simulink model "afe_rst_inv_psm_distributed_control_two_delays"  (R2026a)
settings: Solver=ode1be  StopTime=simlength  FixedStep=tc  MaxStep=Tc
values from neighbouring files (symbols this model uses):
  Amplitude_U = 1.16    [grid_fault_generator.m]
  Amplitude_V = Amplitude_U    (= 1.16)    [grid_fault_generator.m]
  Amplitude_W = Amplitude_U    (= 1.16)    [grid_fault_generator.m]
  end_time_LVRT = start_time_LVRT + error_length    [grid_fault_generator.m]
  Igrid_phase_normalization_factor = 270*sqrt(2)    [grid_emulator.m]
  omega_grid_emulator_nom = w_grid    (= 314.159265359)    [grid_emulator.m]
  omega_grid_nom = w_grid    (= 314.159265359)    [grid_emulator.m]
  t_ramp = 20e-3    (= 0.02)    [grid_fault_generator.m]
  ugrid_factor = 1    [grid_emulator.m]
  V_phase_normalization_factor = Vgrid_phase_normalization_factor    [grid_emulator.m]
  Vdc_bez = 1070    [grid_emulator.m]
  Vemu_ref_norm = Vemu_ref * sqrt(2) / V_phase_normalization_factor    [grid_emulator.m]
  vn_eta_pu = 0    [grid_emulator.m]
  vn_xi_pu = 0    [grid_emulator.m]
  vp_xi_pu = 1    [grid_emulator.m]
undefined symbols (not defined in the file or in its folder): Adrso, Aresd, Bresd, CFi, CFu, Cresd, Crso, CTRPIFF_CLIP_RELEASE, dead_time_INV, emf_fb_p, emf_fb_p_ccaller_1, emf_fb_p_ccaller_2, emf_p, emf_p_ccaller_1, emf_p_ccaller_2, fPWM_INV, g0_161Hz, g0_500Hz, g1_161Hz, g1_500Hz, i_grid_neg_eta_lim, i_grid_neg_eta_red_lim, i_grid_neg_xi_lim, i_grid_neg_xi_red_lim, i_grid_pos_eta_lim, i_grid_pos_eta_red_lim, ibez, id_lim, ieta_neg_ref_lim, ieta_pos_ref_lim, iq_lim, ixi_pos_ref_lim, Jm_norm, k_frt_ref, kg, ki_afe, ki_i, ki_id, ki_iq, ki_rc_neg_grid, ki_rc_pos_grid, ki_vs, ki_w, kp_afe, kp_i, kp_id, kp_iq, kp_rc_neg_grid, kp_rc_pos_grid, kp_vs, kp_w, kw, l1, l2, Lalpha_norm, Ld_norm, Ldrso, Lq_norm, Ls_norm, luenberger_l1 ... (+30)
libraries: fl_lib x146, nesl_utility x62, simulink x8, cstblocks_lti x7, sl_discontinuities x3, single_phase_transformer_lib x3, flexshaft_lib x1, permanent_magnet_synchronous_machine x1
(part 7 of 14)

== system afe_rst_inv_psm_distributed_control_two_delays/INV-Modular/inv_leg_w/driver_board_w/double_integrator_observer ==
  theta : Inport
  Gain : Gain  Gain=kw
  Gain1 : Gain  Gain=kg
  Gain4 : Gain  Gain=omega_bez
  Gain5 : Gain  Gain=ts_inv
  Gain6 : Gain  Gain=1/omega_bez
  Sum : Sum  Inputs=-+|
  Sum1 : Sum  Inputs=|++
  Sum2 : Sum  Inputs=|++
  Sum8 : Sum  Inputs=++|
  Unit Delay1 : UnitDelay  SampleTime=ts_inv
  Unit Delay2 : UnitDelay  SampleTime=ts_inv
  bounder1 : MATLAB Function  TreatAsAtomicUnit=on  SystemSampleTime=ts_inv
  bounder2 : MATLAB Function  TreatAsAtomicUnit=on  SystemSampleTime=ts_inv
  omega_pu_hat : Outport  VectorParamsAs1DForOutWhenUnconnected=off
  theta_hat : Outport  Port=2  VectorParamsAs1DForOutWhenUnconnected=off
  wires:
  theta/1 -> Sum/2  "theta"
  Sum8/1 -> bounder2/1(u)
  Sum1/1 -> Unit Delay2/1
  Unit Delay2/1 -> omega_pu_hat/1, Sum1/2, Gain5/1
  Sum2/1 -> Sum8/2
  bounder2/1(y) -> Unit Delay1/1
  bounder1/1(y) -> Gain/1, Gain1/1
  Gain5/1 -> Gain4/1
  Sum/1 -> bounder1/1(u)
  Unit Delay1/1 -> Sum2/2, theta_hat/1, Sum/1  "theta_hat"
  Gain/1 -> Gain6/1
  Gain6/1 -> Sum1/1
  Gain4/1 -> Sum8/1
  Gain1/1 -> Sum2/1

== system afe_rst_inv_psm_distributed_control_two_delays/INV-Modular/inv_leg_w/driver_board_w/motor_vector_control ==
  motor_torque_ref : Inport
  Bus Creator1 : BusCreator  Inputs=2
  Unit Delay2 : UnitDelay  SampleTime=ts_inv
  Unit Delay3 : UnitDelay  SampleTime=ts_inv
  Variant Source : VariantSource  VariantControls={use_psm_encoder == 1, use_psm_encoder == 0}
  bemf_observer : Subsystem
  current_ctrl : Subsystem
  current_transformation : Subsystem
  dq2alphabeta : MATLAB Function  TreatAsAtomicUnit=on  SystemSampleTime=ts_inv
  us_alphabeta_ctrl : Outport
  tag scope: motor_ualpha_ctrl_dbw=global, motor_ubeta_ctrl_dbw=global
  wires:
  [isv_pu_dbv_fb_dbw] -> current_transformation/2(v)
  Bus Creator1/1 -> us_alphabeta_ctrl/1
  motor_torque_ref/1 -> current_ctrl/1(iq_ref)  "motor_torque_ref"
  dq2alphabeta/2(beta) -> Unit Delay3/1
  [motor_ibeta_pu_dbu] -> bemf_observer/2(ibeta_pu)
  [motor_ubeta_ctrl_dbw] -> Bus Creator1/2  "motor_ubeta_ctrl"
  [isu_pu_dbu_fb_dbw] -> current_transformation/1(u)
  [motor_ualpha_ctrl_dbw] -> Bus Creator1/1  "motor_ualpha_ctrl"
  [motor_ualpha_ctrl_dbu] -> bemf_observer/3(ualpha_pu)
  [motor_ubeta_ctrl_dbu] -> bemf_observer/4(ubeta_pu)
  [motor_ialpha_pu_dbu] -> bemf_observer/1(ialpha_pu)
  current_ctrl/1(ud) -> dq2alphabeta/1(d)
  current_ctrl/2(uq) -> dq2alphabeta/2(q)
  Unit Delay2/1 -> [motor_ualpha_ctrl_dbw]
  [isw_pu_dbw] -> current_transformation/3(w)
  Variant Source/1 -> current_transformation/4(gamma), dq2alphabeta/3(gamma)
  dq2alphabeta/1(alpha) -> Unit Delay2/1
  Unit Delay3/1 -> [motor_ubeta_ctrl_dbw]
  [motor_theta_hat_dbw] -> Variant Source/2
  [motor_phase_mb_fb_dbw_luenberger] -> Variant Source/1

== system afe_rst_inv_psm_distributed_control_two_delays/INV-Modular/inv_leg_w/driver_board_w/voltage-current-acquisition ==
  From3 : From  Commented=on  GotoTag=usu_ctrl_dbu  TagVisibility=global
  From4 : From  Commented=on  GotoTag=usv_ctrl_dbv  TagVisibility=global
  Goto6 : Goto  Commented=on  GotoTag=usu_ctrl_dbu_fb_dbw  TagVisibility=global
  Goto7 : Goto  Commented=on  GotoTag=usv_ctrl_dbv_fb_dbw  TagVisibility=global
  isu_fieldbus : Subsystem
  isv_fieldbus : Subsystem
  isw_measure_and_normalization : Subsystem
  motor_phase_fieldbus : Subsystem
  motor_torque_fieldbus : Subsystem
  usu_ctrl_fieldbus : Subsystem  Commented=on
  usu_fieldbus : Subsystem
  usv_ctrl_fieldbus : Subsystem  Commented=on
  usv_fieldbus : Subsystem
  usw_measure_and_normalization : Subsystem
  tag scope: isu_pu_dbu_fb_dbw=global, isv_pu_dbv_fb_dbw=global, isw_pu_dbw=global, motor_phase_mb_fb_dbw=global, motor_torque_ref_dbu_fb_dbw=global, usu_pu_dbu_fb_dbw=global, usv_pu_dbv_fb_dbw=global, usw_pu_dbw=global
  wires:
  usu_fieldbus/1(us_fb) -> [usu_pu_dbu_fb_dbw]
  usv_fieldbus/1(us_fb) -> [usv_pu_dbv_fb_dbw]
  [usu_pu_dbu] -> usu_fieldbus/1(us)
  [usv_pu_dbv] -> usv_fieldbus/1(us)
  usw_measure_and_normalization/1(us_pu) -> [usw_pu_dbw]
  [usw_dbw] -> usw_measure_and_normalization/1(us)
  isv_fieldbus/1(is_fb) -> [isv_pu_dbv_fb_dbw]
  usv_ctrl_fieldbus/1(u_ctrl_fb) -> Goto7/1
  [isw_dbw] -> isw_measure_and_normalization/1(is)
  From3/1 -> usu_ctrl_fieldbus/1(u_ctrl)
  [isu_pu_dbu] -> isu_fieldbus/1(is)
  isw_measure_and_normalization/1(is_pu) -> [isw_pu_dbw]
  From4/1 -> usv_ctrl_fieldbus/1(u_ctrl)
  isu_fieldbus/1(is_fb) -> [isu_pu_dbu_fb_dbw]
  [isv_pu_dbv] -> isv_fieldbus/1(is)
  usu_ctrl_fieldbus/1(u_ctrl_fb) -> Goto6/1
  motor_torque_fieldbus/1(motor_torque_ref_fb) -> [motor_torque_ref_dbu_fb_dbw]
  [motor_torque_ref_dbu] -> motor_torque_fieldbus/1(motor_torque_ref)
  motor_phase_fieldbus/1(motor_phase_fb) -> [motor_phase_mb_fb_dbw]
  [motor_phase_mb] -> motor_phase_fieldbus/1(motor_phase)

== system afe_rst_inv_psm_distributed_control_two_delays/INV-Modular/inv_leg_w/modulator/sv_pwm ==
  u_alphabeta_ctrl : Inport
  enable : Inport  Port=2
  Bus Selector : BusSelector  OutputSignals=dc
  Bus Selector1 : BusSelector  OutputSignals=motor_ualpha_ctrl,motor_ubeta_ctrl
  C Caller : CCaller  FunctionName=sv_pwm_process_simulink  PortSpecificationStruct="%)30     .    N @   8    (     @         %    \"     4    !     0         %  0 \"0    $    _    07)G3F%M90  4&]R=$YA;64 4V-O<&4     26YD97@     5'EP90      4VEZ90      27-';&]B86P   X    P    !@    @    $          4    (     0    ,    !         !   P!O=70 #@   #     &    \"     0         !0    @    !     P    $         $  # &]U=  .    .     8    (    !          %    \"     $    &     0         0   ...(+2630 chars)"  SampleTime=ts_inv
  Constant : Constant  Value=ts_inv
  Data Type Conversion15 : DataTypeConversion  OutDataTypeStr=single  SaturateOnIntegerOverflow=off  RndMeth=Floor
  Data Type Conversion16 : DataTypeConversion  OutDataTypeStr=single  SaturateOnIntegerOverflow=off  RndMeth=Floor
  Data Type Conversion17 : DataTypeConversion  OutDataTypeStr=uint32  SaturateOnIntegerOverflow=off  RndMeth=Floor
  Data Type Conversion18 : DataTypeConversion  OutDataTypeStr=single  SaturateOnIntegerOverflow=off  RndMeth=Floor
  Data Type Conversion3 : DataTypeConversion  OutDataTypeStr=double  SaturateOnIntegerOverflow=off  RndMeth=Floor
  Zero-Order Hold{,1..3} (4 alike) : ZeroOrderHold  SampleTime=ts_inv
  modulator : Subsystem
  firing_gates : Outport
  wires:
  Bus Selector/1 -> Data Type Conversion3/1  "<dc>"
  Data Type Conversion3/1 -> modulator/1(w)  "dw"
  Bus Selector1/2 -> Data Type Conversion15/1  "<motor_ubeta_ctrl>"
  Bus Selector1/1 -> Data Type Conversion18/1  "<motor_ualpha_ctrl>"
  u_alphabeta_ctrl/1 -> Bus Selector1/1
  modulator/1(firing_gates) -> firing_gates/1
  C Caller/1 -> Bus Selector/1  "out"
  Data Type Conversion15/1 -> Zero-Order Hold1/1
  Zero-Order Hold3/1 -> C Caller/4
  Data Type Conversion17/1 -> Zero-Order Hold3/1
  Zero-Order Hold1/1 -> C Caller/2
  Data Type Conversion16/1 -> Zero-Order Hold2/1
  enable/1 -> Data Type Conversion17/1
  Data Type Conversion18/1 -> Zero-Order Hold/1
  Constant/1 -> Data Type Conversion16/1
  Zero-Order Hold2/1 -> C Caller/3
  Zero-Order Hold/1 -> C Caller/1

== system afe_rst_inv_psm_distributed_control_two_delays/INV-Modular/inv_leg_w/solid_state_inverter/switch_1 ==
  Diode : fl_lib/Electrical/Electrical Elements/Diode  Vf=Vgamma V  Ron=Ron Ohm  Goff=1e-8 1/Ohm  i_specify=off  i_priority=None  i=0 A  i_nominal_specify=off  i_nominal_value=1  i_nominal_unit=A  v_specify=off  v_priority=None  v=0 V  v_nominal_specify=off  v_nominal_value=1  v_nominal_unit=V
  Switch : fl_lib/Electrical/Electrical Elements/Switch  R_closed=Ron Ohm  G_open=1e-8 1/Ohm  Threshold=7.5  i_specify=off  i_priority=None  i=0 A  i_nominal_specify=off  i_nominal_value=1  i_nominal_unit=A  v_specify=off  v_priority=None  v=0 V  v_nominal_specify=off  v_nominal_value=1  v_nominal_unit=V
  snubber : fl_lib/Electrical/Electrical Elements/Capacitor  c=Csnubber F  r=Rsnubber Ohm  g=0 1/Ohm  i_specify=off  i_priority=None  i=0 A  i_nominal_specify=off  i_nominal_value=1  i_nominal_unit=A  v_specify=off  v_priority=None  v=0 V  v_nominal_specify=off  v_nominal_value=1  v_nominal_unit=V  vc_specify=off  vc_priority=High  vc=0 V  vc_nominal_specify=off  vc_nominal_value=1  vc_nominal_unit=V
  G : PMIOPort  Side=Left
  C : PMIOPort  Port=2  Side=Left
  E : PMIOPort  Port=3  Side=Right
  connections:
  Diode/LConn1 -- snubber/RConn1 -- E/RConn1 -- Switch/LConn1
  Switch/RConn1 -- G/RConn1
  Diode/RConn1 -- snubber/LConn1 -- C/RConn1 -- Switch/RConn2

== system afe_rst_inv_psm_distributed_control_two_delays/INV-Modular/inv_leg_w/solid_state_inverter/switch_2 ==
  Diode : fl_lib/Electrical/Electrical Elements/Diode  Vf=Vgamma V  Ron=Ron Ohm  Goff=1e-8 1/Ohm  i_specify=off  i_priority=None  i=0 A  i_nominal_specify=off  i_nominal_value=1  i_nominal_unit=A  v_specify=off  v_priority=None  v=0 V  v_nominal_specify=off  v_nominal_value=1  v_nominal_unit=V
  Switch : fl_lib/Electrical/Electrical Elements/Switch  R_closed=Ron Ohm  G_open=1e-8 1/Ohm  Threshold=7.5  i_specify=off  i_priority=None  i=0 A  i_nominal_specify=off  i_nominal_value=1  i_nominal_unit=A  v_specify=off  v_priority=None  v=0 V  v_nominal_specify=off  v_nominal_value=1  v_nominal_unit=V
  snubber : fl_lib/Electrical/Electrical Elements/Capacitor  c=Csnubber F  r=Rsnubber Ohm  g=0 1/Ohm  i_specify=off  i_priority=None  i=0 A  i_nominal_specify=off  i_nominal_value=1  i_nominal_unit=A  v_specify=off  v_priority=None  v=0 V  v_nominal_specify=off  v_nominal_value=1  v_nominal_unit=V  vc_specify=off  vc_priority=High  vc=0 V  vc_nominal_specify=off  vc_nominal_value=1  vc_nominal_unit=V
  G : PMIOPort  Side=Left
  C : PMIOPort  Port=2  Side=Left
  E : PMIOPort  Port=3  Side=Right
  connections:
  Diode/RConn1 -- snubber/LConn1 -- Switch/RConn2 -- C/RConn1
  Switch/RConn1 -- G/RConn1
  Diode/LConn1 -- snubber/RConn1 -- Switch/LConn1 -- E/RConn1

== system afe_rst_inv_psm_distributed_control_two_delays/grid/grid_emulator/grid_emulator/phase_gen ==
  Constant4 : Constant  Value=omega_grid_emulator_nom
  Integrator : Integrator
  To Workspace7 : ToWorkspace  VariableName=gamma_grid_emulator_sim  SampleTime=ts_afe
      settings: MaxDataPoints=Ns_afe
  bounder1 : MATLAB Function  TreatAsAtomicUnit=on  SystemSampleTime=ts_afe
  grid_emu_phase : Outport  VectorParamsAs1DForOutWhenUnconnected=off
  tag scope: gamma_grid_emulator=global
  wires:
  bounder1/1(y) -> [gamma_grid_emulator], To Workspace7/1, grid_emu_phase/1  "grid_emu_phase"
  Constant4/1 -> Integrator/1
  Integrator/1 -> bounder1/1(u)

== system afe_rst_inv_psm_distributed_control_two_delays/grid/grid_emulator/grid_emulator/voltage_reference ==
  grid_emu_phase : Inport
  Vxi_p : Inport  Port=2
  Vxi_n : Inport  Port=3
  Veta_n : Inport  Port=4
  Constant2 : Constant  Value=0
  Grid: Voltage-Source in abc : Subsystem
  Manual Switch : ManualSwitch  CurrentSetting=0
  Manual Switch1 : ManualSwitch  CurrentSetting=0
  Manual Switch2 : ManualSwitch  CurrentSetting=0
  Sum1 : Sum  Inputs=|++
  Sum4 : Sum  Inputs=|++
  alphabeta2abc : MATLAB Function  TreatAsAtomicUnit=on  SystemSampleTime=ts_afe
  xieta2alphabeta_neg : MATLAB Function  TreatAsAtomicUnit=on  SystemSampleTime=ts_afe
  xieta2alphabeta_pos : MATLAB Function  TreatAsAtomicUnit=on  SystemSampleTime=ts_afe
  V1_ref1 : Outport  VectorParamsAs1DForOutWhenUnconnected=off
  V2_ref1 : Outport  Port=2  VectorParamsAs1DForOutWhenUnconnected=off
  V3_ref1 : Outport  Port=3  VectorParamsAs1DForOutWhenUnconnected=off
  wires:
  xieta2alphabeta_pos/1(alpha) -> Sum1/1
  Sum1/1 -> alphabeta2abc/1(alpha)
  xieta2alphabeta_pos/2(beta) -> Sum4/1
  Sum4/1 -> alphabeta2abc/2(beta)
  xieta2alphabeta_neg/1(alpha) -> Sum1/2
  xieta2alphabeta_neg/2(beta) -> Sum4/2
  grid_emu_phase/1 -> Grid: Voltage-Source in abc/1(gamma), xieta2alphabeta_neg/3(gamma), xieta2alphabeta_pos/3(gamma)
  Vxi_p/1 -> xieta2alphabeta_pos/1(xi)
  Constant2/1 -> xieta2alphabeta_pos/2(eta)
  Vxi_n/1 -> xieta2alphabeta_neg/1(xi)
  Veta_n/1 -> xieta2alphabeta_neg/2(eta)
  alphabeta2abc/1(a) -> [V1_ref_xieta]
  alphabeta2abc/2(b) -> [V2_ref_xieta]
  alphabeta2abc/3(c) -> [V3_ref_xieta]
  [V3_ref_abc] -> Manual Switch2/2
  Manual Switch2/1 -> V3_ref1/1
  [V2_ref_abc] -> Manual Switch1/2
  Manual Switch/1 -> V1_ref1/1
  Grid: Voltage-Source in abc/1(vp_xi) -> [V1_ref_abc]
  Grid: Voltage-Source in abc/2(vn_xi) -> [V2_ref_abc]
  Grid: Voltage-Source in abc/3(vn_eta) -> [V3_ref_abc]
  [V1_ref_abc] -> Manual Switch/2
  [V1_ref_xieta] -> Manual Switch/1
  [V2_ref_xieta] -> Manual Switch1/1
  Manual Switch1/1 -> V2_ref1/1
  [V3_ref_xieta] -> Manual Switch2/1

== system afe_rst_inv_psm_distributed_control_two_delays/grid/grid_emulator/grid_emulator/voltage_source ==
  Constant : Constant  Value=vp_xi_pu
  Constant1 : Constant  Value=vn_xi_pu
  Constant2 : Constant  Value=vn_eta_pu
  Gain1 : Gain  Gain=V_phase_normalization_factor
  Gain2 : Gain  Gain=ugrid_factor
  Gain3 : Gain  Gain=ugrid_factor
  Gain4 : Gain  Gain=ugrid_factor
  Gain7 : Gain  Gain=V_phase_normalization_factor
  Gain8 : Gain  Gain=V_phase_normalization_factor
  LTI System3 : cstblocks_lti/LTI System  sys=LVRT_flt_ss_c  IC=[]  PadeOrder=0
  LTI System4 : cstblocks_lti/LTI System  sys=LVRT_flt_ss_c  IC=[]  PadeOrder=0
  LTI System5 : cstblocks_lti/LTI System  sys=LVRT_flt_ss_c  IC=[]  PadeOrder=0
  vp_xi : Outport  VectorParamsAs1DForOutWhenUnconnected=off
  vn_xi : Outport  Port=2  VectorParamsAs1DForOutWhenUnconnected=off
  vn_eta : Outport  Port=3  VectorParamsAs1DForOutWhenUnconnected=off
  wires:
  LTI System3/1 -> Gain7/1
  LTI System4/1 -> Gain8/1
  Gain7/1 -> Gain2/1
  Gain8/1 -> Gain3/1
  Gain1/1 -> Gain4/1
  LTI System5/1 -> Gain1/1
  Gain2/1 -> vp_xi/1
  Gain3/1 -> vn_xi/1
  Gain4/1 -> vn_eta/1
  Constant2/1 -> LTI System5/1
  Constant1/1 -> LTI System4/1
  Constant/1 -> LTI System3/1

== system afe_rst_inv_psm_distributed_control_two_delays/grid/instantaneus_power/abc2alphabeta/abc2alphabeta ==
  a : Inport
  b : Inport  Port=2
  c : Inport  Port=3
  Gain1 : Gain  Gain=-1/2
  Gain11 : Gain  Gain=-1/2
  Gain2 : Gain  Gain=0
  Gain3 : Gain  Gain=sqrt(3)/2
  Gain4 : Gain  Gain=-sqrt(3)/2
  Gain8 : Gain  Gain=2/3
  Gain9 : Gain  Gain=2/3
  Sum : Sum  Inputs=+++
  Sum1 : Sum  Inputs=+++
  "alpha " : Outport  VectorParamsAs1DForOutWhenUnconnected=off
  "beta " : Outport  Port=2  VectorParamsAs1DForOutWhenUnconnected=off
  wires:
  Gain11/1 -> Sum/2
  Gain1/1 -> Sum/3
  Gain9/1 -> "beta "/1
  Gain8/1 -> "alpha "/1
  Gain2/1 -> Sum1/1
  Gain3/1 -> Sum1/2
  Gain4/1 -> Sum1/3
  a/1 -> Gain2/1, Sum/1
  c/1 -> Gain4/1, Gain1/1
  b/1 -> Gain3/1, Gain11/1
  Sum/1 -> Gain8/1
  Sum1/1 -> Gain9/1

== system afe_rst_inv_psm_distributed_control_two_delays/grid/instantaneus_power/abc2alphabeta /abc->alphabeta ==
  a : Inport
  b : Inport  Port=2
  c : Inport  Port=3
  Gain1 : Gain  Gain=-1/2
  Gain11 : Gain  Gain=-1/2
  Gain2 : Gain  Gain=0
  Gain3 : Gain  Gain=sqrt(3)/2
  Gain4 : Gain  Gain=-sqrt(3)/2
  Gain8 : Gain  Gain=2/3
  Gain9 : Gain  Gain=2/3
  Sum : Sum  Inputs=+++
  Sum1 : Sum  Inputs=+++
  "alpha " : Outport  VectorParamsAs1DForOutWhenUnconnected=off
  "beta " : Outport  Port=2  VectorParamsAs1DForOutWhenUnconnected=off
  wires:
  Sum1/1 -> Gain9/1
  Sum/1 -> Gain8/1
  b/1 -> Gain11/1, Gain3/1
  c/1 -> Gain1/1, Gain4/1
  a/1 -> Sum/1, Gain2/1
  Gain4/1 -> Sum1/3
  Gain3/1 -> Sum1/2
  Gain2/1 -> Sum1/1
  Gain8/1 -> "alpha "/1
  Gain9/1 -> "beta "/1
  Gain1/1 -> Sum/3
  Gain11/1 -> Sum/2

== system afe_rst_inv_psm_distributed_control_two_delays/mainboard_afe/current_sequence_avg/Moving Average Filter5/Enabled Subsystem ==
  In1 : Inport
  Enable : EnablePort
  Constant2 : Constant
  Divide : Product  Inputs=*/
  Gain1 : Gain  Gain=1/(2*pi)
  Gain9 : Gain  Gain=2
  Zero-Order Hold : ZeroOrderHold  SampleTime=ts_afe
  Out1 : Outport
  wires:
  Gain1/1 -> Gain9/1
  Zero-Order Hold/1 -> Out1/1  "period"
  Gain9/1 -> Divide/2
  In1/1 -> Gain1/1  "Omega_el"
  Divide/1 -> Zero-Order Hold/1
  Constant2/1 -> Divide/1

== system afe_rst_inv_psm_distributed_control_two_delays/mainboard_afe/current_sequence_avg/Moving Average Filter5/Reset Trigger ==
  Clock : Clock
  Constant1 : Constant  Value=simlength
  Constant3 : Constant  Value=0
  Constant4 : Constant
  Mod : Math  Operator=mod
  Switch : Switch  Criteria=u2 ~= 0  SaturateOnIntegerOverflow=off  InputSameDT=off
  Zero-Order Hold : ZeroOrderHold  SampleTime=ts_afe
  Out1 : Outport
  wires:
  Constant1/1 -> Mod/2
  Switch/1 -> Out1/1  "Reset"
  Clock/1 -> Zero-Order Hold/1
  Mod/1 -> Switch/2
  Constant4/1 -> Switch/3
  Zero-Order Hold/1 -> Mod/1
  Constant3/1 -> Switch/1

== system afe_rst_inv_psm_distributed_control_two_delays/mainboard_afe/current_sequence_avg/Moving Average Filter6/Enabled Subsystem ==
  In1 : Inport
  Enable : EnablePort
  Constant2 : Constant
  Divide : Product  Inputs=*/
  Gain1 : Gain  Gain=1/(2*pi)
  Gain9 : Gain  Gain=2
  Zero-Order Hold : ZeroOrderHold  SampleTime=ts_afe
  Out1 : Outport
  wires:
  Constant2/1 -> Divide/1
  Divide/1 -> Zero-Order Hold/1
  In1/1 -> Gain1/1  "Omega_el"
  Gain9/1 -> Divide/2
  Zero-Order Hold/1 -> Out1/1  "period"
  Gain1/1 -> Gain9/1

== system afe_rst_inv_psm_distributed_control_two_delays/mainboard_afe/current_sequence_avg/Moving Average Filter6/Reset Trigger ==
  Clock : Clock
  Constant1 : Constant  Value=simlength
  Constant3 : Constant  Value=0
  Constant4 : Constant
  Mod : Math  Operator=mod
  Switch : Switch  Criteria=u2 ~= 0  SaturateOnIntegerOverflow=off  InputSameDT=off
  Zero-Order Hold : ZeroOrderHold  SampleTime=ts_afe
  Out1 : Outport
  wires:
  Constant3/1 -> Switch/1
  Zero-Order Hold/1 -> Mod/1
  Constant4/1 -> Switch/3
  Mod/1 -> Switch/2
  Clock/1 -> Zero-Order Hold/1
  Switch/1 -> Out1/1  "Reset"
  Constant1/1 -> Mod/2

== system afe_rst_inv_psm_distributed_control_two_delays/mainboard_afe/current_sequence_avg/Moving Average Filter7/Enabled Subsystem ==
  In1 : Inport
  Enable : EnablePort
  Constant2 : Constant
  Divide : Product  Inputs=*/
  Gain1 : Gain  Gain=1/(2*pi)
  Gain9 : Gain  Gain=2
  Zero-Order Hold : ZeroOrderHold  SampleTime=ts_afe
  Out1 : Outport
  wires:
  Gain1/1 -> Gain9/1
  Zero-Order Hold/1 -> Out1/1  "period"
  Gain9/1 -> Divide/2
  In1/1 -> Gain1/1  "Omega_el"
  Divide/1 -> Zero-Order Hold/1
  Constant2/1 -> Divide/1

== system afe_rst_inv_psm_distributed_control_two_delays/mainboard_afe/current_sequence_avg/Moving Average Filter7/Reset Trigger ==
  Clock : Clock
  Constant1 : Constant  Value=simlength
  Constant3 : Constant  Value=0
  Constant4 : Constant
  Mod : Math  Operator=mod
  Switch : Switch  Criteria=u2 ~= 0  SaturateOnIntegerOverflow=off  InputSameDT=off
  Zero-Order Hold : ZeroOrderHold  SampleTime=ts_afe
  Out1 : Outport
  wires:
  Constant1/1 -> Mod/2
  Switch/1 -> Out1/1  "Reset"
  Clock/1 -> Zero-Order Hold/1
  Mod/1 -> Switch/2
  Constant4/1 -> Switch/3
  Zero-Order Hold/1 -> Mod/1
  Constant3/1 -> Switch/1

== system afe_rst_inv_psm_distributed_control_two_delays/mainboard_afe/current_sequence_avg/Moving Average Filter8/Enabled Subsystem ==
  In1 : Inport
  Enable : EnablePort
  Constant2 : Constant
  Divide : Product  Inputs=*/
  Gain1 : Gain  Gain=1/(2*pi)
  Gain9 : Gain  Gain=2
  Zero-Order Hold : ZeroOrderHold  SampleTime=ts_afe
  Out1 : Outport
  wires:
  Constant2/1 -> Divide/1
  Divide/1 -> Zero-Order Hold/1
  In1/1 -> Gain1/1  "Omega_el"
  Gain9/1 -> Divide/2
  Zero-Order Hold/1 -> Out1/1  "period"
  Gain1/1 -> Gain9/1

== system afe_rst_inv_psm_distributed_control_two_delays/mainboard_afe/current_sequence_avg/Moving Average Filter8/Reset Trigger ==
  Clock : Clock
  Constant1 : Constant  Value=simlength
  Constant3 : Constant  Value=0
  Constant4 : Constant
  Mod : Math  Operator=mod
  Switch : Switch  Criteria=u2 ~= 0  SaturateOnIntegerOverflow=off  InputSameDT=off
  Zero-Order Hold : ZeroOrderHold  SampleTime=ts_afe
  Out1 : Outport
  wires:
  Constant3/1 -> Switch/1
  Zero-Order Hold/1 -> Mod/1
  Constant4/1 -> Switch/3
  Mod/1 -> Switch/2
  Clock/1 -> Zero-Order Hold/1
  Switch/1 -> Out1/1  "Reset"
  Constant1/1 -> Mod/2

== system afe_rst_inv_psm_distributed_control_two_delays/mainboard_afe/dq_pll/pll_stageA/abc_to_alphabeta ==
  ug_a : Inport
  ug_b : Inport  Port=2
  ug_c : Inport  Port=3
  abc2alphabeta : MATLAB Function  TreatAsAtomicUnit=on  SystemSampleTime=ts_afe
  ug_alpha : Outport  VectorParamsAs1DForOutWhenUnconnected=off
  ug_beta : Outport  Port=2  VectorParamsAs1DForOutWhenUnconnected=off
  wires:
  abc2alphabeta/2(beta) -> ug_beta/1  "u_grid_beta"
  abc2alphabeta/1(alpha) -> ug_alpha/1  "u_grid_alpha"
  ug_c/1 -> abc2alphabeta/3(c)
  ug_b/1 -> abc2alphabeta/2(b)
  ug_a/1 -> abc2alphabeta/1(a)

== system afe_rst_inv_psm_distributed_control_two_delays/mainboard_afe/dq_pll/pll_stageA/sequences ==
  u_grid_alpha : Inport
  u_grid_beta : Inport  Port=2
  gamma_grid : Inport  Port=3
  alphabeta2xieta : Subsystem
  u_grid_pos_xi : Outport
  u_grid_pos_eta : Outport  Port=2
  wires:
  alphabeta2xieta/1(xi) -> u_grid_pos_xi/1  "u_grid_pos_xi"
  alphabeta2xieta/2(eta) -> u_grid_pos_eta/1  "u_grid_pos_eta"
  u_grid_alpha/1 -> alphabeta2xieta/1(alpha)  "u_grid_alpha"
  u_grid_beta/1 -> alphabeta2xieta/2(beta)  "u_grid_beta"
  gamma_grid/1 -> alphabeta2xieta/3(gamma)  "gamma_grid"

== system afe_rst_inv_psm_distributed_control_two_delays/mainboard_afe/dq_pll/pll_stageB/double_integrator_observer ==
  theta : Inport
  Gain : Gain  Gain=Ldrso  Multiplication=Matrix(K*u)
  Gain1 : Gain  Gain=Adrso  Multiplication=Matrix(K*u)
  Gain2 : Gain  Gain=Crso  Multiplication=Matrix(K*u)
  Selector : Selector  InputPortWidth=2  IndexOptions=Index vector (dialog)  Indices=2  OutputSizes=1
  Sum : Sum  Inputs=-+|
  Sum1 : Sum  Inputs=|++
  Unit Delay : UnitDelay  SampleTime=ts_afe
  Zero-Order Hold : ZeroOrderHold  SampleTime=ts_afe
  bounder1 : MATLAB Function  TreatAsAtomicUnit=on  SystemSampleTime=ts_afe
  bounder2 : MATLAB Function  TreatAsAtomicUnit=on  SystemSampleTime=ts_afe
  omega_hat : Outport
  wires:
  Gain/1 -> Sum1/1
  Selector/1 -> omega_hat/1
  Gain2/1 -> bounder2/1(u)  "theta_hat"
  Gain1/1 -> Sum1/2
  Sum1/1 -> Unit Delay/1
  Sum/1 -> bounder1/1(u)  "e"
  Unit Delay/1 -> Gain1/1, Selector/1, Gain2/1
  theta/1 -> Zero-Order Hold/1  "theta"
  Zero-Order Hold/1 -> Sum/2  "theta_dsp"
  bounder1/1(y) -> Gain/1  "e_bounded"
  bounder2/1(y) -> Sum/1  "theta_hat_bounded"

== system afe_rst_inv_psm_distributed_control_two_delays/mainboard_afe/voltage_sequence_avg/Moving Average Filter1/Enabled Subsystem ==
  In1 : Inport
  Enable : EnablePort
  Constant2 : Constant
  Divide : Product  Inputs=*/
  Gain1 : Gain  Gain=1/(2*pi)
  Gain9 : Gain  Gain=2
  Zero-Order Hold : ZeroOrderHold  SampleTime=ts_afe
  Out1 : Outport
  wires:
  Gain1/1 -> Gain9/1
  Zero-Order Hold/1 -> Out1/1  "period"
  Gain9/1 -> Divide/2
  In1/1 -> Gain1/1  "Omega_el"
  Divide/1 -> Zero-Order Hold/1
  Constant2/1 -> Divide/1

== system afe_rst_inv_psm_distributed_control_two_delays/mainboard_afe/voltage_sequence_avg/Moving Average Filter1/Reset Trigger ==
  Clock : Clock
  Constant1 : Constant  Value=simlength
  Constant3 : Constant  Value=0
  Constant4 : Constant
  Mod : Math  Operator=mod
  Switch : Switch  Criteria=u2 ~= 0  SaturateOnIntegerOverflow=off  InputSameDT=off
  Zero-Order Hold : ZeroOrderHold  SampleTime=ts_afe
  Out1 : Outport
  wires:
  Constant1/1 -> Mod/2
  Switch/1 -> Out1/1  "Reset"
  Clock/1 -> Zero-Order Hold/1
  Mod/1 -> Switch/2
  Constant4/1 -> Switch/3
  Zero-Order Hold/1 -> Mod/1
  Constant3/1 -> Switch/1

== system afe_rst_inv_psm_distributed_control_two_delays/mainboard_afe/voltage_sequence_avg/Moving Average Filter2/Enabled Subsystem ==
  In1 : Inport
  Enable : EnablePort
  Constant2 : Constant
  Divide : Product  Inputs=*/
  Gain1 : Gain  Gain=1/(2*pi)
  Gain9 : Gain  Gain=2
  Zero-Order Hold : ZeroOrderHold  SampleTime=ts_afe
  Out1 : Outport
  wires:
  Constant2/1 -> Divide/1
  Divide/1 -> Zero-Order Hold/1
  In1/1 -> Gain1/1  "Omega_el"
  Gain9/1 -> Divide/2
  Zero-Order Hold/1 -> Out1/1  "period"
  Gain1/1 -> Gain9/1

== system afe_rst_inv_psm_distributed_control_two_delays/mainboard_afe/voltage_sequence_avg/Moving Average Filter2/Reset Trigger ==
  Clock : Clock
  Constant1 : Constant  Value=simlength
  Constant3 : Constant  Value=0
  Constant4 : Constant
  Mod : Math  Operator=mod
  Switch : Switch  Criteria=u2 ~= 0  SaturateOnIntegerOverflow=off  InputSameDT=off
  Zero-Order Hold : ZeroOrderHold  SampleTime=ts_afe
  Out1 : Outport
  wires:
  Constant3/1 -> Switch/1
  Zero-Order Hold/1 -> Mod/1
  Constant4/1 -> Switch/3
  Mod/1 -> Switch/2
  Clock/1 -> Zero-Order Hold/1
  Switch/1 -> Out1/1  "Reset"
  Constant1/1 -> Mod/2

== system afe_rst_inv_psm_distributed_control_two_delays/mainboard_afe/voltage_sequence_avg/Moving Average Filter3/Enabled Subsystem ==
  In1 : Inport
  Enable : EnablePort
  Constant2 : Constant
  Divide : Product  Inputs=*/
  Gain1 : Gain  Gain=1/(2*pi)
  Gain9 : Gain  Gain=2
  Zero-Order Hold : ZeroOrderHold  SampleTime=ts_afe
  Out1 : Outport
  wires:
  Gain1/1 -> Gain9/1
  Zero-Order Hold/1 -> Out1/1  "period"
  Gain9/1 -> Divide/2
  In1/1 -> Gain1/1  "Omega_el"
  Divide/1 -> Zero-Order Hold/1
  Constant2/1 -> Divide/1

== system afe_rst_inv_psm_distributed_control_two_delays/mainboard_afe/voltage_sequence_avg/Moving Average Filter3/Reset Trigger ==
  Clock : Clock
  Constant1 : Constant  Value=simlength
  Constant3 : Constant  Value=0
  Constant4 : Constant
  Mod : Math  Operator=mod
  Switch : Switch  Criteria=u2 ~= 0  SaturateOnIntegerOverflow=off  InputSameDT=off
  Zero-Order Hold : ZeroOrderHold  SampleTime=ts_afe
  Out1 : Outport
  wires:
  Constant1/1 -> Mod/2
  Switch/1 -> Out1/1  "Reset"
  Clock/1 -> Zero-Order Hold/1
  Mod/1 -> Switch/2
  Constant4/1 -> Switch/3
  Zero-Order Hold/1 -> Mod/1
  Constant3/1 -> Switch/1

== system afe_rst_inv_psm_distributed_control_two_delays/mainboard_afe/voltage_sequence_avg/Moving Average Filter4/Enabled Subsystem ==
  In1 : Inport
  Enable : EnablePort
  Constant2 : Constant
  Divide : Product  Inputs=*/
  Gain1 : Gain  Gain=1/(2*pi)
  Gain9 : Gain  Gain=2
  Zero-Order Hold : ZeroOrderHold  SampleTime=ts_afe
  Out1 : Outport
  wires:
  Constant2/1 -> Divide/1
  Divide/1 -> Zero-Order Hold/1
  In1/1 -> Gain1/1  "Omega_el"
  Gain9/1 -> Divide/2
  Zero-Order Hold/1 -> Out1/1  "period"
  Gain1/1 -> Gain9/1

== system afe_rst_inv_psm_distributed_control_two_delays/mainboard_afe/voltage_sequence_avg/Moving Average Filter4/Reset Trigger ==
  Clock : Clock
  Constant1 : Constant  Value=simlength
  Constant3 : Constant  Value=0
  Constant4 : Constant
  Mod : Math  Operator=mod
  Switch : Switch  Criteria=u2 ~= 0  SaturateOnIntegerOverflow=off  InputSameDT=off
  Zero-Order Hold : ZeroOrderHold  SampleTime=ts_afe
  Out1 : Outport
  wires:
  Constant3/1 -> Switch/1
  Zero-Order Hold/1 -> Mod/1
  Constant4/1 -> Switch/3
  Mod/1 -> Switch/2
  Clock/1 -> Zero-Order Hold/1
  Switch/1 -> Out1/1  "Reset"
  Constant1/1 -> Mod/2

== system afe_rst_inv_psm_distributed_control_two_delays/AFE-Modular/afe_leg_a/driver_board_a/current_ctrl/phase_current_control ==
  In1 : Inport
  is_abc : Inport  Port=2
  Bus Creator1 : BusCreator  Inputs=2
  Bus Creator2 : BusCreator  Inputs=3
  Bus Selector1 : BusSelector  OutputSignals=usa_ctrl,usb_ctrl,usc_ctrl
  MATLAB Function : MATLAB Function  TreatAsAtomicUnit=on
  Selector : Selector  InputPortWidth=3  IndexOptions=Index vector (dialog)  Indices=1  OutputSizes=1
  Unit Delay2 : UnitDelay  SampleTime=ts_afe
  Unit Delay3 : UnitDelay  SampleTime=ts_afe
  isa_ref/isa : Scope  NumInputPorts=2
      settings: SampleTime=ts_afe  ActiveDisplayYMinimum=-1.14664  ActiveDisplayYMaximum=1.21003
  phase-current-control-dba : Subsystem
  us_alphabeta_ctrl : Outport  VectorParamsAs1DForOutWhenUnconnected=off
  tag scope: usa_ctrl_dba=global
  wires:
  Bus Creator1/1 -> us_alphabeta_ctrl/1
  Unit Delay2/1 -> Bus Creator1/1  "us_alpha_ctrl"
  Bus Selector1/1 -> MATLAB Function/1(a)  "<usa_ctrl>"
  MATLAB Function/2(beta) -> Unit Delay3/1
  Bus Selector1/2 -> MATLAB Function/2(b)  "<usb_ctrl>"
  Unit Delay3/1 -> Bus Creator1/2  "us_beta_ctrl"
  MATLAB Function/1(alpha) -> Unit Delay2/1
  Bus Selector1/3 -> MATLAB Function/3(c)  "<usc_ctrl>"
  phase-current-control-dba/1(Out1) -> [usa_ctrl_dba], Bus Creator2/1  "usa_ctrl"
  is_abc/1 -> phase-current-control-dba/2(is_abc), isa_ref/isa/2  "isa"
  In1/1 -> Selector/1
  [usb_ctrl_dbb_fb_dba] -> Bus Creator2/2  "usb_ctrl"
  [usc_ctrl_dbc_fb_dba] -> Bus Creator2/3  "usc_ctrl"
  Bus Creator2/1 -> Bus Selector1/1  "us_abc_ctrl"
  Selector/1 -> phase-current-control-dba/1(In1), isa_ref/isa/1  "isa_ref"

== system afe_rst_inv_psm_distributed_control_two_delays/AFE-Modular/afe_leg_a/driver_board_a/current_ctrl/xieta2abc ==
  pos_xi : Inport
  pos_eta : Inport  Port=2
  neg_xi : Inport  Port=3
  neg_eta : Inport  Port=4
  gamma : Inport  Port=5
  MATLAB Function2 : MATLAB Function  TreatAsAtomicUnit=on
  Mux : Mux  Inputs=3
  Negative Sequence : MATLAB Function  TreatAsAtomicUnit=on
  Positive Sequence : MATLAB Function  TreatAsAtomicUnit=on
  Sum : Sum  Inputs=|++
  Sum1 : Sum  Inputs=|++
  i_abc : Outport
  wires:
  Mux/1 -> i_abc/1  "i_abc"
  pos_eta/1 -> Positive Sequence/2(eta)
  pos_xi/1 -> Positive Sequence/1(xi)
  neg_xi/1 -> Negative Sequence/1(xi)
  Sum1/1 -> MATLAB Function2/2(beta)
  MATLAB Function2/2(b) -> Mux/2  "i_b"
  Negative Sequence/2(beta) -> Sum1/2
  Positive Sequence/1(alpha) -> Sum/1
  Negative Sequence/1(alpha) -> Sum/2
  MATLAB Function2/3(c) -> Mux/3  "i_c"
  gamma/1 -> Positive Sequence/3(gamma), Negative Sequence/3(gamma)
  Sum/1 -> MATLAB Function2/1(alpha)
  Positive Sequence/2(beta) -> Sum1/1
  MATLAB Function2/1(a) -> Mux/1  "i_a"
  neg_eta/1 -> Negative Sequence/2(eta)

== system afe_rst_inv_psm_distributed_control_two_delays/AFE-Modular/afe_leg_a/driver_board_a/dq_pll/pll_stageA ==
  gamma_grid : Inport
  Math Function : Math  Operator=magnitude^2  SignedPower=on
  Math Function1 : Math  Operator=magnitude^2  SignedPower=on
  Reciprocal Sqrt : Sqrt  Operator=rSqrt
  Saturation : Saturate  UpperLimit=inf  LowerLimit=0.02
  Sum : Sum  Inputs=|++
  sequences : Subsystem
  transformation : Subsystem
  u_grid_pos_xi : Outport  VectorParamsAs1DForOutWhenUnconnected=off
  u_grid_pos_eta : Outport  Port=2  VectorParamsAs1DForOutWhenUnconnected=off
  tag scope: ugrid_unorm_phase_a=global
  wires:
  transformation/1(ug_alpha) -> Math Function/1, sequences/1(u_grid_alpha)
  transformation/2(ug_beta) -> Math Function1/1, sequences/2(u_grid_beta)
  Math Function/1 -> Sum/1
  Math Function1/1 -> Sum/2
  Sum/1 -> Saturation/1
  Reciprocal Sqrt/1 -> [ugrid_unorm_phase_a]
  Saturation/1 -> Reciprocal Sqrt/1
  gamma_grid/1 -> sequences/3(gamma_grid)
  sequences/1(u_grid_pos_xi) -> u_grid_pos_xi/1
  sequences/2(u_grid_pos_eta) -> u_grid_pos_eta/1
  [ugb_pu_dbb_fb_dba] -> transformation/2(ug_b)
  [uga_pu_dba] -> transformation/1(ug_a)
  [ugc_pu_dbc_fb_dba] -> transformation/3(ug_c)

== system afe_rst_inv_psm_distributed_control_two_delays/AFE-Modular/afe_leg_a/driver_board_a/dq_pll/pll_stageB ==
  u_grid_pos_xi : Inport
  u_grid_pos_eta : Inport  Port=2
  -2<x<2 : Saturate  UpperLimit=2  LowerLimit=-2
  Constant4 : Constant  Value=omega_grid_nom
  Product1 : Product  RndMeth=Zero
  Product2 : Product  RndMeth=Zero
  Sum3 : Sum  SaturateOnIntegerOverflow=on
  Sum4 : Sum  SaturateOnIntegerOverflow=on
  Sum5 : Sum  Inputs=++|
  Unit Delay{1..5} (5 alike) : UnitDelay  SampleTime=ts_afe
  bounder1 : MATLAB Function  TreatAsAtomicUnit=on  SystemSampleTime=ts_afe
  kp : Gain  Gain=pll_i1*ts_afe  SaturateOnIntegerOverflow=on  OutDataTypeStr=Inherit: Same as input  ParamDataTypeStr=Inherit: Same as input
  kp1 : Gain  Gain=pll_p  SaturateOnIntegerOverflow=on  OutDataTypeStr=Inherit: Same as input  ParamDataTypeStr=Inherit: Same as input
  kp2 : Gain  Gain=ts_afe  SaturateOnIntegerOverflow=on  OutDataTypeStr=Inherit: Same as input  ParamDataTypeStr=Inherit: Same as input
  gamma_grid_pll : Outport  VectorParamsAs1DForOutWhenUnconnected=off
  wires:
  Unit Delay4/1 -> Sum5/2, Sum3/2
  Sum3/1 -> -2<x<2/1
  Sum4/1 -> bounder1/1(u)
  Unit Delay1/1 -> Sum4/2
  -2<x<2/1 -> Unit Delay4/1  "i1"
  kp2/1 -> Sum4/1
  Constant4/1 -> Product2/2
  [ugrid_unorm_phase_a] -> Unit Delay3/1
  kp/1 -> Sum3/1
  Sum5/1 -> Product2/1
  bounder1/1(y) -> Unit Delay1/1, Unit Delay2/1
  u_grid_pos_eta/1 -> Unit Delay5/1
  Product2/1 -> kp2/1
  Product1/1 -> kp/1, kp1/1  "V l"
  kp1/1 -> Sum5/1
  Unit Delay2/1 -> gamma_grid_pll/1
  Unit Delay3/1 -> Product1/2
  Unit Delay5/1 -> Product1/1

== system afe_rst_inv_psm_distributed_control_two_delays/AFE-Modular/afe_leg_a/driver_board_a/voltage-current-acquisition/is_eta_neg_ref_fieldbus ==
  is : Inport
  Unit Delay : UnitDelay  SampleTime=ts_afe
  Unit Delay1 : UnitDelay  SampleTime=ts_afe
  Zero-Order Hold : ZeroOrderHold  SampleTime=ts_afe
  is_fb : Outport
  wires:
  is/1 -> Zero-Order Hold/1
  Unit Delay/1 -> Unit Delay1/1
  Zero-Order Hold/1 -> Unit Delay/1
  Unit Delay1/1 -> is_fb/1

== system afe_rst_inv_psm_distributed_control_two_delays/AFE-Modular/afe_leg_a/driver_board_a/voltage-current-acquisition/is_eta_pos_ref_fieldbus ==
  is : Inport
  Unit Delay : UnitDelay  SampleTime=ts_afe
  Unit Delay1 : UnitDelay  SampleTime=ts_afe
  Zero-Order Hold : ZeroOrderHold  SampleTime=ts_afe
  is_fb : Outport
  wires:
  is/1 -> Zero-Order Hold/1
  Unit Delay/1 -> Unit Delay1/1
  Zero-Order Hold/1 -> Unit Delay/1
  Unit Delay1/1 -> is_fb/1

== system afe_rst_inv_psm_distributed_control_two_delays/AFE-Modular/afe_leg_a/driver_board_a/voltage-current-acquisition/is_xi_neg_ref_fieldbus ==
  is : Inport
  Unit Delay : UnitDelay  SampleTime=ts_afe
  Unit Delay1 : UnitDelay  SampleTime=ts_afe
  Zero-Order Hold : ZeroOrderHold  SampleTime=ts_afe
  is_fb : Outport
  wires:
  Unit Delay/1 -> Unit Delay1/1
  Zero-Order Hold/1 -> Unit Delay/1
  is/1 -> Zero-Order Hold/1
  Unit Delay1/1 -> is_fb/1

== system afe_rst_inv_psm_distributed_control_two_delays/AFE-Modular/afe_leg_a/driver_board_a/voltage-current-acquisition/isa_measure ==
  is : Inport
  Gain : Gain  Gain=1/Igrid_phase_normalization_factor
  Quantizer : Quantizer  QuantizationInterval=CurrentQuantization
  Unit Delay : UnitDelay  SampleTime=ts_afe
  Zero-Order Hold : ZeroOrderHold  SampleTime=ts_afe
  is_pu : Outport
  wires:
  Quantizer/1 -> Zero-Order Hold/1
  Gain/1 -> is_pu/1
  Zero-Order Hold/1 -> Unit Delay/1
  Unit Delay/1 -> Gain/1
  is/1 -> Quantizer/1

== system afe_rst_inv_psm_distributed_control_two_delays/AFE-Modular/afe_leg_a/driver_board_a/voltage-current-acquisition/isb_fieldbus ==
  is : Inport
  Unit Delay : UnitDelay  SampleTime=ts_afe
  Unit Delay1 : UnitDelay  SampleTime=ts_afe
  Zero-Order Hold : ZeroOrderHold  SampleTime=ts_afe
  is_fb : Outport
  wires:
  is/1 -> Zero-Order Hold/1
  Unit Delay/1 -> Unit Delay1/1
  Zero-Order Hold/1 -> Unit Delay/1
  Unit Delay1/1 -> is_fb/1

== system afe_rst_inv_psm_distributed_control_two_delays/AFE-Modular/afe_leg_a/driver_board_a/voltage-current-acquisition/isc_fieldbus ==
  is : Inport
  Unit Delay : UnitDelay  SampleTime=ts_afe
  Unit Delay1 : UnitDelay  SampleTime=ts_afe
  Zero-Order Hold : ZeroOrderHold  SampleTime=ts_afe
  is_fb : Outport
  wires:
  is/1 -> Zero-Order Hold/1
  Unit Delay/1 -> Unit Delay1/1
  Zero-Order Hold/1 -> Unit Delay/1
  Unit Delay1/1 -> is_fb/1

== system afe_rst_inv_psm_distributed_control_two_delays/AFE-Modular/afe_leg_a/driver_board_a/voltage-current-acquisition/ixi_ref_fieldbus ==
  is : Inport
  Unit Delay : UnitDelay  SampleTime=ts_afe
  Unit Delay1 : UnitDelay  SampleTime=ts_afe
  Zero-Order Hold : ZeroOrderHold  SampleTime=ts_afe
  is_fb : Outport
  wires:
  is/1 -> Zero-Order Hold/1
  Unit Delay/1 -> Unit Delay1/1
  Zero-Order Hold/1 -> Unit Delay/1
  Unit Delay1/1 -> is_fb/1

== system afe_rst_inv_psm_distributed_control_two_delays/AFE-Modular/afe_leg_a/driver_board_a/voltage-current-acquisition/ixi_ref_fieldbus1 ==
  is : Inport
  Unit Delay : UnitDelay  SampleTime=ts_afe
  Unit Delay1 : UnitDelay  SampleTime=ts_afe
  Zero-Order Hold : ZeroOrderHold  SampleTime=ts_afe
  is_fb : Outport
  wires:
  is/1 -> Zero-Order Hold/1
  Unit Delay/1 -> Unit Delay1/1
  Zero-Order Hold/1 -> Unit Delay/1
  Unit Delay1/1 -> is_fb/1

== system afe_rst_inv_psm_distributed_control_two_delays/AFE-Modular/afe_leg_a/driver_board_a/voltage-current-acquisition/ub_ctrl_fieldbus ==
  u_ctrl : Inport
  Unit Delay : UnitDelay  SampleTime=ts_afe
  Unit Delay1 : UnitDelay  SampleTime=ts_afe
  Zero-Order Hold : ZeroOrderHold  SampleTime=ts_afe
  u_ctrl_fb : Outport
  wires:
  u_ctrl/1 -> Zero-Order Hold/1
  Unit Delay/1 -> Unit Delay1/1
  Zero-Order Hold/1 -> Unit Delay/1
  Unit Delay1/1 -> u_ctrl_fb/1

== system afe_rst_inv_psm_distributed_control_two_delays/AFE-Modular/afe_leg_a/driver_board_a/voltage-current-acquisition/uc_ctrl_fieldbus ==
  u_ctrl : Inport
  Unit Delay : UnitDelay  SampleTime=ts_afe
  Unit Delay1 : UnitDelay  SampleTime=ts_afe
  Zero-Order Hold : ZeroOrderHold  SampleTime=ts_afe
  u_ctrl_fb : Outport
  wires:
  Zero-Order Hold/1 -> Unit Delay/1
  u_ctrl/1 -> Zero-Order Hold/1
  Unit Delay/1 -> Unit Delay1/1
  Unit Delay1/1 -> u_ctrl_fb/1

== system afe_rst_inv_psm_distributed_control_two_delays/AFE-Modular/afe_leg_a/driver_board_a/voltage-current-acquisition/uga_measure ==
  ug : Inport
  Gain : Gain  Gain=1/V_phase_normalization_factor
  Quantizer : Quantizer  QuantizationInterval=CurrentQuantization
  Unit Delay : UnitDelay  SampleTime=ts_afe
  Zero-Order Hold : ZeroOrderHold  SampleTime=ts_afe
  ug_pu : Outport
  wires:
  ug/1 -> Quantizer/1
  Unit Delay/1 -> Gain/1
  Zero-Order Hold/1 -> Unit Delay/1
  Gain/1 -> ug_pu/1
  Quantizer/1 -> Zero-Order Hold/1

== system afe_rst_inv_psm_distributed_control_two_delays/AFE-Modular/afe_leg_a/driver_board_a/voltage-current-acquisition/ugb_fieldbus ==
  ug : Inport
  Unit Delay : UnitDelay  SampleTime=ts_afe
  Unit Delay1 : UnitDelay  SampleTime=ts_afe
  Zero-Order Hold : ZeroOrderHold  SampleTime=ts_afe
  ug_fb : Outport
  wires:
  ug/1 -> Zero-Order Hold/1
  Zero-Order Hold/1 -> Unit Delay/1
  Unit Delay/1 -> Unit Delay1/1
  Unit Delay1/1 -> ug_fb/1

== system afe_rst_inv_psm_distributed_control_two_delays/AFE-Modular/afe_leg_a/driver_board_a/voltage-current-acquisition/ugc_fieldbus ==
  ug : Inport
  Unit Delay : UnitDelay  SampleTime=ts_afe
  Unit Delay1 : UnitDelay  SampleTime=ts_afe
  Zero-Order Hold : ZeroOrderHold  SampleTime=ts_afe
  ug_fb : Outport
  wires:
  ug/1 -> Zero-Order Hold/1
  Unit Delay/1 -> Unit Delay1/1
  Zero-Order Hold/1 -> Unit Delay/1
  Unit Delay1/1 -> ug_fb/1

== system afe_rst_inv_psm_distributed_control_two_delays/AFE-Modular/afe_leg_a/modulator/sv_pwm/modulator ==
  u : Inport
  v : Inport  Port=2
  w : Inport  Port=3
  Bus Creator : BusCreator  Inputs=6
  PWM generator 1 : Subsystem  mask{f=fPWM_INV, ph=0, m_up=0.98, m_low=0.02, dead_time=dead_time_INV, vg_firing=15, polarity=1}
      mask prompts: f "Frequency"; ph "Phase"; m_up "Max Input Modulation Value"; m_low "Min Input Modulation Value"; dead_time "Dead Time"; vg_firing "Gate Voltage"
  PWM generator 2 : Subsystem  mask{f=fPWM_INV, ph=0, m_up=0.98, m_low=0.02, dead_time=dead_time_INV, vg_firing=15, polarity=1}
      mask prompts: f "Frequency"; ph "Phase"; m_up "Max Input Modulation Value"; m_low "Min Input Modulation Value"; dead_time "Dead Time"; vg_firing "Gate Voltage"
  PWM generator 3 : Subsystem  mask{f=fPWM_INV, ph=0, m_up=0.98, m_low=0.02, dead_time=dead_time_INV, vg_firing=15, polarity=1}
      mask prompts: f "Frequency"; ph "Phase"; m_up "Max Input Modulation Value"; m_low "Min Input Modulation Value"; dead_time "Dead Time"; vg_firing "Gate Voltage"
  firing_gates : Outport
  wires:
  u/1 -> PWM generator 1/1(m_index)
  w/1 -> PWM generator 3/1(m_index)
  v/1 -> PWM generator 2/1(m_index)
  PWM generator 1/2(m2) -> Bus Creator/2  "pwm_u_bottom"
  Bus Creator/1 -> firing_gates/1
  PWM generator 2/1(m1) -> Bus Creator/3  "pwm_v_top"
  PWM generator 3/1(m1) -> Bus Creator/5  "pwm_w_top"
  PWM generator 2/2(m2) -> Bus Creator/4  "pwm_v_bottom"
  PWM generator 3/2(m2) -> Bus Creator/6  "pwm_w_bottom"
  PWM generator 1/1(m1) -> Bus Creator/1  "pwm_u_top"

== system afe_rst_inv_psm_distributed_control_two_delays/AFE-Modular/afe_leg_b/driver_board_b/current_ctrl/phase_current_control ==
  In1 : Inport
  is_abc : Inport  Port=2
  Bus Creator1 : BusCreator  Inputs=2
  Bus Creator2 : BusCreator  Inputs=3
  Bus Selector1 : BusSelector  OutputSignals=usa_ctrl,usb_ctrl,usc_ctrl
  MATLAB Function : MATLAB Function  TreatAsAtomicUnit=on
  Selector : Selector  InputPortWidth=3  IndexOptions=Index vector (dialog)  Indices=2  OutputSizes=1
  Unit Delay2 : UnitDelay  SampleTime=ts_afe
  Unit Delay3 : UnitDelay  SampleTime=ts_afe
  isb_ref/isb : Scope  NumInputPorts=2
      settings: SampleTime=ts_afe  ActiveDisplayYMinimum=-2.19741  ActiveDisplayYMaximum=6.15124
  phase-current-control-dbb : Subsystem
  us_alphabeta_ctrl : Outport  VectorParamsAs1DForOutWhenUnconnected=off
  tag scope: usb_ctrl_dbb=global
  wires:
  Bus Creator1/1 -> us_alphabeta_ctrl/1
  Unit Delay2/1 -> Bus Creator1/1  "us_alpha_ctrl"
  Bus Selector1/1 -> MATLAB Function/1(a)  "<usa_ctrl>"
  MATLAB Function/2(beta) -> Unit Delay3/1
  Bus Selector1/2 -> MATLAB Function/2(b)  "<usb_ctrl>"
  Unit Delay3/1 -> Bus Creator1/2  "us_beta_ctrl"
  MATLAB Function/1(alpha) -> Unit Delay2/1
  Bus Selector1/3 -> MATLAB Function/3(c)  "<usc_ctrl>"
  is_abc/1 -> phase-current-control-dbb/2(is_abc), isb_ref/isb/2  "isb"
  In1/1 -> Selector/1
  [usc_ctrl_dbc_fb_dbb] -> Bus Creator2/3  "usc_ctrl"
  phase-current-control-dbb/1(Out1) -> [usb_ctrl_dbb], Bus Creator2/2  "usb_ctrl"
  [usa_ctrl_dba_fb_dbb] -> Bus Creator2/1  "usa_ctrl"
  Bus Creator2/1 -> Bus Selector1/1  "us_abc_ctrl"
  Selector/1 -> phase-current-control-dbb/1(In1), isb_ref/isb/1  "isb_ref"

== system afe_rst_inv_psm_distributed_control_two_delays/AFE-Modular/afe_leg_b/driver_board_b/current_ctrl/xieta2abc ==
  pos_xi : Inport
  pos_eta : Inport  Port=2
  neg_xi : Inport  Port=3
  neg_eta : Inport  Port=4
  gamma : Inport  Port=5
  MATLAB Function2 : MATLAB Function  TreatAsAtomicUnit=on
  Mux : Mux  Inputs=3
  Negative Sequence : MATLAB Function  TreatAsAtomicUnit=on
  Positive Sequence : MATLAB Function  TreatAsAtomicUnit=on
  Sum : Sum  Inputs=|++
  Sum1 : Sum  Inputs=|++
  i_abc_reference : Outport
  wires:
  Mux/1 -> i_abc_reference/1  "i_abc_reference"
  pos_eta/1 -> Positive Sequence/2(eta)
  pos_xi/1 -> Positive Sequence/1(xi)
  neg_xi/1 -> Negative Sequence/1(xi)
  Sum1/1 -> MATLAB Function2/2(beta)
  MATLAB Function2/2(b) -> Mux/2  "i_b"
  Negative Sequence/2(beta) -> Sum1/2
  Positive Sequence/1(alpha) -> Sum/1
  Negative Sequence/1(alpha) -> Sum/2
  MATLAB Function2/3(c) -> Mux/3  "i_c"
  gamma/1 -> Positive Sequence/3(gamma), Negative Sequence/3(gamma)
  Sum/1 -> MATLAB Function2/1(alpha)
  Positive Sequence/2(beta) -> Sum1/1
  MATLAB Function2/1(a) -> Mux/1  "i_a"
  neg_eta/1 -> Negative Sequence/2(eta)

== system afe_rst_inv_psm_distributed_control_two_delays/AFE-Modular/afe_leg_b/driver_board_b/dq_pll/pll_stageA ==
  gamma_grid : Inport
  Math Function : Math  Operator=magnitude^2  SignedPower=on
  Math Function1 : Math  Operator=magnitude^2  SignedPower=on
  Reciprocal Sqrt : Sqrt  Operator=rSqrt
  Saturation : Saturate  UpperLimit=inf  LowerLimit=0.02
  Sum : Sum  Inputs=|++
  mormalization_and_transformation : Subsystem
  sequences : Subsystem
  u_grid_pos_xi : Outport  VectorParamsAs1DForOutWhenUnconnected=off
  u_grid_pos_eta : Outport  Port=2  VectorParamsAs1DForOutWhenUnconnected=off
  tag scope: ugrid_unorm_phase_b=global
  wires:
  mormalization_and_transformation/1(ug_alpha) -> Math Function/1, sequences/1(u_grid_alpha)
  mormalization_and_transformation/2(ug_beta) -> Math Function1/1, sequences/2(u_grid_beta)
  Math Function/1 -> Sum/1
  Math Function1/1 -> Sum/2
  Sum/1 -> Saturation/1
  Reciprocal Sqrt/1 -> [ugrid_unorm_phase_b]
  Saturation/1 -> Reciprocal Sqrt/1
  gamma_grid/1 -> sequences/3(gamma_grid)
  sequences/1(u_grid_pos_xi) -> u_grid_pos_xi/1
  sequences/2(u_grid_pos_eta) -> u_grid_pos_eta/1
  [ugb_pu_dbb] -> mormalization_and_transformation/2(ug_b)
  [uga_pu_dba_fb_dbb] -> mormalization_and_transformation/1(ug_a)
  [ugc_pu_dbc_fb_dbb] -> mormalization_and_transformation/3(ug_c)
